simulink model "residual_FWD_INV_validation"  (R2025a)
settings: Solver=VariableStepAuto  StartTime=0.0  StopTime=375  RelTol=1e-3
undefined symbols (not defined in the file or in its folder): National_Instruments, PCI, shadowInverseOptions, shadowOptions, shadowPressureOptions, singlePassOptions
libraries: sldrtlib x3
(part 2 of 2)

== matlab function residual_FWD_INV_validation/MATLAB Function8 ==
  settings: updateMethod=DISCRETE  sampleTime=0.05
  data: inverseContext input Bus: ResidualShadowContextBus size=1; desiredMotion input size=[6 1]; desiredPressurePrediction_bar output double; nominalPressurePrediction_bar output double; desiredPressureDiagnostic output Bus: ResidualSinglePassDiagnosticsBus size=1; shadowPressureOptions input; variableCommon input; singlePassOptions input
function [desiredPressurePrediction_bar,nominalPressurePrediction_bar,desiredPressureDiagnostic]= ...
    rlResidualDesiredPressureBlock(inverseContext,desiredMotion, ...
    shadowPressureOptions,variableCommon,singlePassOptions) %#ok<INUSD>
%RLRESIDUALDESIREDPRESSUREBLOCK Paste into a discrete 0.05 s MATLAB Function.
% desiredMotion = [l2d;l3d;dl2d;dl3d;ddl2d;ddl3d], double 6x1, SI units.
% Feedforward pressure for DESIRED motion, with a frozen observed residual.
% One GRU evaluation at actual measured q/v, actual command and causal history.
% No recurrent-state update, inverse iterations or integration in this block.
% This is a single-pass inverse approximation, not an exact nonlinear solve.
% Initial installation: Scopes/logging only; existing valve/Kill wiring stays.
% Diagnostic output type: Bus: ResidualSinglePassDiagnosticsBus (unchanged).
% variableCommon is retained for port compatibility and is not used.
% Pressure options: 4=min(0), 5=max, 8=slew, 9=activation(0), 10=N/bar.
%#codegen
desiredPressurePrediction_bar=nan(3,1);nominalPressurePrediction_bar=nan(3,1);
desiredPressureDiagnostic=residualSinglePassDiagnostics();
assert(isequal(size(desiredMotion),[6 1]),'desiredMotion must be a 6x1 column.');
if ~inverseContext.valid,return;end
assert(all(isfinite(singlePassOptions))&& ...
    (singlePassOptions(1)==64||singlePassOptions(1)==128)&&singlePassOptions(2)>0);
assert(singlePassOptions(1)==inverseContext.units);
if ~all(isfinite([inverseContext.measured;inverseContext.pressure_bar; ...
        inverseContext.historyPre;inverseContext.featureDt_s;inverseContext.horizon_s; ...
        inverseContext.sampleTime_host_s;desiredMotion])) || ...
        inverseContext.featureDt_s<=0 || inverseContext.horizon_s<=0
    return;
end
assert(all(isfinite(shadowPressureOptions([4;5;8;9;10]))));
assert(shadowPressureOptions(4)==0,'Collection policy requires zero minimum pressure.');
assert(shadowPressureOptions(9)==0,'Use the as-trained zero-activation pressure map.');
maximum=shadowPressureOptions(5);slew=shadowPressureOptions(8);alpha=shadowPressureOptions(10);
assert(maximum>0&&slew>0&&alpha>0);
network=residualControllerNetwork(singlePassOptions(1));
assert(abs(alpha-network.forcePerBar)<1e-10*network.forcePerBar);
if any(inverseContext.pressure_bar<-1e-9)||any(inverseContext.pressure_bar>maximum+1e-9),return;end
physics=residualShadowPhysicsConfig();n=physics.nominal;
% Both branches target precisely the SAME desired trajectory.
qd=desiredMotion(1:2);vd=desiredMotion(3:4);ad=desiredMotion(5:6);
P=forceResidualPhysics(qd,vd,n);M=[P(1),P(2);P(2),P(3)];C=[P(4),P(5);P(6),P(7)];
target=M*ad+(C+n.D)*vd+n.K*qd+ ...
    armS_single_boundForce(qd,n.mu,n.lKbounds)+P(8:9);
if ~all(isfinite(target)),return;end
% History and GRU features remain ACTUAL observations, not desired motion.
[~,residual]=residualGruCell(network,[inverseContext.measured; ...
    inverseContext.pressure_bar;inverseContext.featureDt_s],inverseContext.historyPre);
desiredPressureDiagnostic.networkEvaluations=uint8(1);
request=target-residual;
[corrected,allocationLimited]=minimumPressure(request,alpha,maximum);
[nominal,nominalLimited]=minimumPressure(target,alpha,maximum);
step=slew*inverseContext.horizon_s;
p=min(max(corrected,inverseContext.pressure_bar-step),inverseContext.pressure_bar+step);
pn=min(max(nominal,inverseContext.pressure_bar-step),inverseContext.pressure_bar+step);
if ~all(isfinite([target;residual;corrected;nominal;p;pn])),return;end
B=alpha*[-1 1 0;-1 0 1];
desiredPressurePrediction_bar=p;nominalPressurePrediction_bar=pn;
desiredPressureDiagnostic.valid=true;
desiredPressureDiagnostic.allocationLimited=allocationLimited;
desiredPressureDiagnostic.slewLimited=any(abs(p-corrected)>1e-9);
desiredPressureDiagnostic.nominalAllocationLimited=nominalLimited;
desiredPressureDiagnostic.nominalSlewLimited=any(abs(pn-nominal)>1e-9);
desiredPressureDiagnostic.targetForce_N=target;desiredPressureDiagnostic.residualForce_N=residual;
desiredPressureDiagnostic.correctedForceRequest_N=request;
desiredPressureDiagnostic.frozenTotalForce_N=B*p+residual;
desiredPressureDiagnostic.allocationError_N=B*corrected-request;
desiredPressureDiagnostic.slewError_N=B*(p-corrected);
desiredPressureDiagnostic.frozenBalanceError_N=B*p+residual-target;
desiredPressureDiagnostic.nominalBalanceError_N=B*pn-target;
desiredPressureDiagnostic.frozenBalanceSatisfied=norm(desiredPressureDiagnostic.frozenBalanceError_N)<=singlePassOptions(2);
desiredPressureDiagnostic.residualInputPressure_bar=inverseContext.pressure_bar;
desiredPressureDiagnostic.correctedPressureBeforeSlew_bar=corrected;
desiredPressureDiagnostic.nominalPressureBeforeSlew_bar=nominal;
desiredPressureDiagnostic.pressureDifferenceBeforeSlew_bar=corrected-nominal;
desiredPressureDiagnostic.pressureDifference_bar=p-pn;
desiredPressureDiagnostic.sampleTime_host_s=inverseContext.sampleTime_host_s;
desiredPressureDiagnostic.horizon_s=inverseContext.horizon_s;
end
function [pressure,limited]=minimumPressure(force,alpha,maximum)
forceBar=force/alpha;p1=max([0;-forceBar(1);-forceBar(2)]);
pressure=max([p1;p1+forceBar(1);p1+forceBar(2)],0);
peak=max(pressure);limited=peak>maximum;
if limited,pressure=pressure*(maximum/peak);end
pressure(pressure<=1e-8)=0;
end

== matlab function residual_FWD_INV_validation/Seperate paramter calculation/MATLAB Function ==
  data: u input; theta output; phi output
function [theta, phi] = length2config(u)
%#codegen
% This file convert the length changes into theta/phi
%
% Inputs:
%   u       : length change[2x1] (m)
%             [l2; l3]
%
% Outputs:
%   theta   : bending direction [constant] (rad)
%   phi     : bending amount [constant] (rad)

l = [0.0; u(1); u(2)];
r  = 0.013;

c = [atan2(l(3) - l(2), sqrt(0.3e1) * (l(2) + l(3)));
    0.2e1 / 0.3e1 / r * sqrt((3 * l(2) ^ 2 + 3 * l(3) * l(2) + 3 * l(3) ^ 2))];

theta = c(1);
phi = c(2);

end

== matlab function residual_FWD_INV_validation/Seperate paramter calculation/MATLAB Function2 ==
  data: u input; l output
function l = lengthVector(u)
%#codegen
% This file create the length vector
%
% Inputs:
%   u       : length change[2x1] (m)
%             [l2; l3]
%
% Outputs:
%   l   : bending direction [3x1] (m)

l = [-(u(1) + u(2)); u(1); u(2)];

end

== matlab function residual_FWD_INV_validation/NDI Sensor reading/Position Hold ==
  data: u input; y output
function y = fcn(u)
persistent lastPosition
if isempty(lastPosition), lastPosition=nan(3,1); end
if all(isfinite(u)), lastPosition=u; end
y=lastPosition;
end

== matlab function residual_FWD_INV_validation/NDI Sensor reading/Sensor/MATLAB Function ==
  data: x input; xx output; y input; z input; yy output; zz output
function [xx,yy,zz] = rotateX90(x,y,z)

    R = [1 0 0;
         0 0 1;
         0 -1 0];

    p = R*[x;y;z]*0.001;

    xx=p(1);
    yy=p(2);
    zz=p(3);

    
end

== matlab function residual_FWD_INV_validation/NDI Sensor reading/Sensor/MATLAB Function2 ==
  data: rel_p input; theta output; phi output; phi_prev input; residual output; valid output
function [theta,phi,residual,valid] = xyz2ThetaPhi(rel_p,phi_prev)
persistent lastPhi lastTheta lastOutputTheta lastOutputPhi lastResidual
if isempty(lastPhi)
    lastPhi=0.0001; lastTheta=0;
    lastOutputTheta=NaN; lastOutputPhi=NaN; lastResidual=NaN;
end
% Keep the external memory for compatibility; never use its NaN.
if isfinite(phi_prev), lastPhi=phi_prev; end
[theta,phi,residual,valid]=ndiSupportFnc.configuration(rel_p,lastPhi,lastTheta);
if valid
    lastPhi=phi; lastTheta=theta;
    lastOutputTheta=theta; lastOutputPhi=phi; lastResidual=residual;
else
    % Scope outputs hold, but configurationValid remains false.
    theta=lastOutputTheta; phi=lastOutputPhi; residual=lastResidual;
end
end

== matlab function residual_FWD_INV_validation/MATLAB Function3 ==
  data: l input; pressure_bar output; tauDesired_N output; tauAvailable_N output; limited output; modelValid output; orientationValid input; stiff input
function [pressure_bar, tauDesired_N, tauAvailable_N, limited, modelValid] = ...
    rlInverseModelBlock(l, orientationValid, stiff)
%#codegen
% Paste-ready replacement for the collection inverseModel MATLAB Function.
% Keeps the existing 3 inputs / 5 outputs, invalid hold and allocation policy.
% Requires the corrected armS_single_boundForce.m on the MATLAB path.
% Bound value remains +/-0.035 m; no SLX edited or hardware run.
% l = [l2;l3;dl2;dl3;ddl2;ddl3], SI units.
% Invalid input/model evaluation holds the last successful outputs.
% modelValid=false identifies held outputs.
% Persistent values reset when the block is initialized for a new run.
% stiff remains unused, matching the original implementation.

persistent lastPressure lastTauDesired lastTauAvailable lastLimited

if isempty(lastPressure)
    lastPressure = zeros(3,1);
    lastTauDesired = zeros(2,1);
    lastTauAvailable = zeros(2,1);
    lastLimited = false;
end

% Default to the last successful outputs.
pressure_bar = lastPressure;
tauDesired_N = lastTauDesired;
tauAvailable_N = lastTauAvailable;
limited = lastLimited;
modelValid = false;

if ~orientationValid || ~all(isfinite(l(:)))
    return;
end

q = l(1:2);
dq = l(3:4);
ddq = l(5:6);

params.N = 1;
params.L = 0.17411;
params.r = 0.013;
params.mi = 0.1;
params.g = [0;0;-9.81];
params.K = 650*[2 1;1 2];
% params.K = stiff * [2 1;1 2];
params.D = 40*eye(2);
params.mu = 2000;
params.lKbounds = [-0.035;0.035;1e6];

[M,C,G] = armS_single_core(q,dq,params);

if ~all(isfinite(M(:))) || ~all(isfinite(C(:))) || ...
        ~all(isfinite(G(:)))
    return;
end

% Equal soft bounds on all three actuator lengths, including l1=-l2-l3.
bound = armS_single_boundForce(q,params.mu,params.lKbounds);
tauCandidate = M*ddq + (C+params.D)*dq + G + params.K*q + bound;
if ~all(isfinite(tauCandidate(:)))
    return;
end

forcePerBar = pi*(params.r/2)^2*1e5;
forceBar = tauCandidate/forcePerBar;
p1 = max([0;-forceBar(1);-forceBar(2)]);
effective = max([p1;p1+forceBar(1);p1+forceBar(2)],0);

deadzone_bar = 0.0;
maxCommand_bar = 3.0;
maxEffective_bar = maxCommand_bar-deadzone_bar;

limitedCandidate = false;
peak = max(effective);
if peak > maxEffective_bar
    effective = effective*(maxEffective_bar/peak);
    limitedCandidate = true;
end

pressureCandidate = zeros(3,1);
for i = 1:3
    if effective(i) > 1e-8
        pressureCandidate(i) = effective(i)+deadzone_bar;
    end
end

availableCandidate = ...
    forcePerBar*[-1 1 0;-1 0 1]*effective;

if ~all(isfinite(pressureCandidate(:))) || ...
        ~all(isfinite(availableCandidate(:)))
    return;
end

% Commit only a successful calculation.
lastPressure = pressureCandidate;
lastTauDesired = tauCandidate;
lastTauAvailable = availableCandidate;
lastLimited = limitedCandidate;

pressure_bar = lastPressure;
tauDesired_N = lastTauDesired;
tauAvailable_N = lastTauAvailable;
limited = lastLimited;
modelValid = true;
end

== matlab function residual_FWD_INV_validation/NDI Sensor reading/Sensor/MATLAB Function1 ==
  data: sensorRelativeXYZ_m input; moduleTipXYZ_m output; R_NDI_from_arm input; theta input; phi input; orientationValid input; baseOrientationValid input; tipXYZValid output
function [moduleTipXYZ_m,tipXYZValid] = moduleTipXYZBlock( ...
    sensorRelativeXYZ_m,R_NDI_from_arm,theta,phi, ...
    orientationValid,baseOrientationValid)
%#codegen
% Input XYZ: existing Sensor/position output, metres, AFTER rotateX90.
% Output XYZ: physical module endpoint relative to module base, expressed
% in the CURRENT calibrated module-base frame. Not world-frame position.
% Assumes axial sensor mounting offsets: base .055 m, distal .050 m.
moduleTipXYZ_m=nan(3,1);
tipXYZValid=false;
if ~orientationValid || ~baseOrientationValid || ...
        ~all(isfinite(sensorRelativeXYZ_m(:))) || ...
        ~all(isfinite(R_NDI_from_arm(:))) || ...
        ~isfinite(theta) || ~isfinite(phi)
    return;
end
if norm(R_NDI_from_arm.'*R_NDI_from_arm-eye(3),'fro')>1e-3 || ...
        abs(det(R_NDI_from_arm)-1)>1e-3
    return;
end
% Undo the legacy fixed plotting-frame rotation, then use measured base pose.
R_fixed=[1 0 0;0 0 1;0 -1 0];
sensorXYZ_arm=R_NDI_from_arm.'*R_fixed.'*sensorRelativeXYZ_m(:);
% Measured tip tangent reconstructed from orientation-derived theta/phi.
% This does not reconstruct XYZ from a constant-curvature arc.
tipTangent=[sin(phi)*cos(theta);sin(phi)*sin(theta);cos(phi)];
moduleTipXYZ_m=sensorXYZ_arm-[0;0;0.055]-0.050*tipTangent;
tipXYZValid=true;
end
